simulink model "gm_HFMA_4B_1_5_9_13"  (R2026b)
settings: Solver=FixedStepDiscrete  StopTime=stopTime  FixedStep=1.953125e-06
PreLoadFcn:
  | load('a_luts.mat')
undefined symbols (not defined in the file or in its folder): Ts
libraries: simulink x202, simulink_need_slupdate x99, hdlsllib x91
(part 2 of 20)

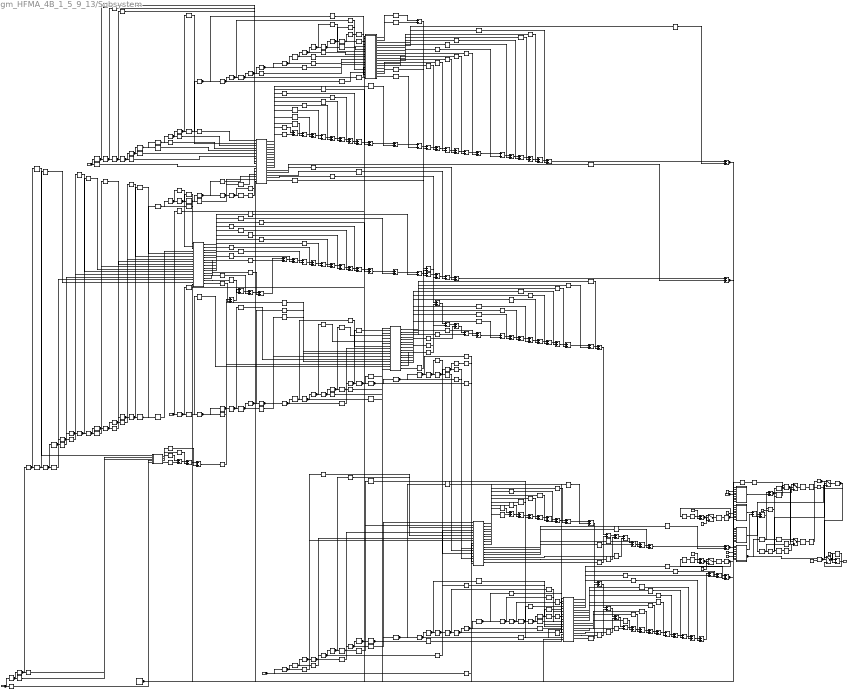
== system gm_HFMA_4B_1_5_9_13/Subsystem ==
  note: U(k)
  note: U(k)
  note: Latches the Output
  Mic1 : Inport  OutDataTypeStr=fixdt(1, 16, 15)  PortDimensions=1  SampleTime=0.000125
  Mic2 : Inport  Port=2  OutDataTypeStr=fixdt(1, 16, 15)  PortDimensions=1  SampleTime=0.000125
  Mic3 : Inport  Port=3  OutDataTypeStr=fixdt(1, 16, 15)  PortDimensions=1  SampleTime=0.000125
  Mic4 : Inport  Port=4  OutDataTypeStr=fixdt(1, 16, 15)  PortDimensions=1  SampleTime=0.000125
  RESET : Inport  Port=5  OutDataTypeStr=boolean  PortDimensions=1  SampleTime=0.000125
  Add{,25,27,29} (4 alike) : Sum  OutDataTypeStr=fixdt(1, 20, 17)  AccumDataTypeStr=fixdt(1, 22, 27)  SaturateOnIntegerOverflow=on  SampleTime=1.953125e-06
  Add{1,21,110,113,115,211..213} (8 alike) : Sum  OutDataTypeStr=fixdt(1, 20, 17)  AccumDataTypeStr=fixdt(1, 30, 26)  SaturateOnIntegerOverflow=on  SampleTime=1.953125e-06
  Add{7,10,12,15,71..73,101..103,121..123,151..153} (16 alike) : Sum  OutDataTypeStr=fixdt(1, 20, 17)  AccumDataTypeStr=fixdt(1, 24, 20)  SaturateOnIntegerOverflow=on  SampleTime=1.953125e-06
  Add{11,111..112,114} (4 alike) : Sum  OutDataTypeStr=fixdt(1, 20, 17)  AccumDataTypeStr=fixdt(1, 21, 17)  SaturateOnIntegerOverflow=on  SampleTime=1.953125e-06
  Add{9,13,91..93,131..133} (8 alike) : Sum  OutDataTypeStr=fixdt(1, 20, 17)  AccumDataTypeStr=fixdt(1, 23, 19)  SaturateOnIntegerOverflow=on  SampleTime=1.953125e-06
  Add{5,8,14,17,51..53,81..83,141..143,171..173} (16 alike) : Sum  OutDataTypeStr=fixdt(1, 20, 17)  AccumDataTypeStr=fixdt(1, 25, 21)  SaturateOnIntegerOverflow=on  SampleTime=1.953125e-06
  Add{2,6,16,20,24,26,28,61..63,161..163,201..203} (16 alike) : Sum  OutDataTypeStr=fixdt(1, 20, 17)  AccumDataTypeStr=fixdt(1, 27, 23)  SaturateOnIntegerOverflow=on  SampleTime=1.953125e-06
  Add{4,18,41..43,181..183} (8 alike) : Sum  OutDataTypeStr=fixdt(1, 20, 17)  AccumDataTypeStr=fixdt(1, 26, 22)  SaturateOnIntegerOverflow=on  SampleTime=1.953125e-06
  Add{3,19,22,31..33,191..193,221..223} (12 alike) : Sum  OutDataTypeStr=fixdt(1, 20, 17)  AccumDataTypeStr=fixdt(1, 28, 24)  SaturateOnIntegerOverflow=on  SampleTime=1.953125e-06
  Add{23,231..233} (4 alike) : Sum  OutDataTypeStr=fixdt(1, 20, 17)  AccumDataTypeStr=fixdt(1, 31, 27)  SaturateOnIntegerOverflow=on  SampleTime=1.953125e-06
  Add_stage2 : Sum  OutDataTypeStr=fixdt(0, 42, 34)  AccumDataTypeStr=fixdt(0, 42, 34)  SaturateOnIntegerOverflow=on  SampleTime=1.953125e-06
  Add_stage3 : Sum  OutDataTypeStr=fixdt(0, 42, 34)  AccumDataTypeStr=fixdt(0, 42, 34)  SaturateOnIntegerOverflow=on  SampleTime=1.953125e-06
  Add_stage4 : Sum  OutDataTypeStr=fixdt(0, 40, 34)  AccumDataTypeStr=fixdt(0, 42, 34)  SaturateOnIntegerOverflow=on  SampleTime=1.953125e-06
  Compare : RelationalOperator  Operator=<=  OutDataTypeStr=boolean  SampleTime=1.953125e-06
  Compare1 : RelationalOperator  Operator===  OutDataTypeStr=boolean  SampleTime=0.000125
  Constant : Constant  Value=0  OutDataTypeStr=uint8  SampleTime=1.953125e-06
  Constant1 : Constant  OutDataTypeStr=fixdt(0, 18, 0)  SampleTime=1.953125e-06
  Constant13 : Constant  Value=13  OutDataTypeStr=fixdt(0, 18, 0)  SampleTime=1.953125e-06
  Constant2 : Constant  Value=0  OutDataTypeStr=uint8  SampleTime=1.953125e-06
  Constant3 : Constant  Value=0  OutDataTypeStr=uint8  SampleTime=1.953125e-06
  Constant4 : Constant  Value=90  OutDataTypeStr=fixdt(0, 18, 11)  SampleTime=0.000125
  Constant5 : Constant  Value=5  OutDataTypeStr=fixdt(0, 18, 0)  SampleTime=1.953125e-06
  Constant6 : Constant  Value=180  OutDataTypeStr=uint8  SampleTime=0.000125
  Constant9 : Constant  Value=9  OutDataTypeStr=fixdt(0, 18, 0)  SampleTime=1.953125e-06
  Delay{,1..24,31..34,41..43,51..53,61..63,71..73,81..83,91..93,101..103,111..114,121..124,131..134,141..144,151..153,161..163,171..173,181..183,191..193,201..203,211..214,221..224,231..234} (96 alike) : Delay  DelayLength=1  InitialCondition=0  SampleTime=0.000125
  Delay110 : RateTransition  OutPortSampleTimeOpt=Multiple of input port sample time  OutPortSampleTimeMultiple=64
  Delay1_absorbed : Delay  DelayLength=0
  Delay25 : RateTransition  OutPortSampleTimeOpt=Multiple of input port sample time  OutPortSampleTimeMultiple=64
  Delay3_bypass : Delay  DelayLength=1  InitialCondition=0  SampleTime=0.000125
  Delay3_lowered : Delay  DelayLength=1  InitialCondition=0  SampleTime=0.000125
  Delay_Switch : Switch  Criteria=u2 ~= 0  OutDataTypeStr=uint8  SampleTime=0.000125  SaturateOnIntegerOverflow=off  InputSameDT=off
  Delay_absorbed : Delay  DelayLength=0
  FixPt Constant : Constant  OutDataTypeStr=uint8  SampleTime=1.953125e-06
  FixPt Constant1 : Constant  OutDataTypeStr=uint8  SampleTime=1.953125e-06
  FixPt Sum1 : Sum  OutDataTypeStr=uint8  AccumDataTypeStr=uint8  SampleTime=1.953125e-06
  FixPt Sum11 : Sum  OutDataTypeStr=uint8  AccumDataTypeStr=uint8  SampleTime=1.953125e-06
  FixPt Switch : Switch  Criteria=u2 > Threshold  Threshold="fi(0,0,8,0,\"hex\",\"27\")"  OutDataTypeStr=uint8  SampleTime=1.953125e-06  SaturateOnIntegerOverflow=off  InputSameDT=off
  FixPt Switch1 : Switch  Criteria=u2 > Threshold  Threshold="fi(0,0,8,0,\"hex\",\"b4\")"  OutDataTypeStr=uint8  SampleTime=1.953125e-06  SaturateOnIntegerOverflow=off  InputSameDT=off
  Force to be scalar : SignalSpecification  OutDataTypeStr=uint8  Dimensions=1
  Force to be scalar1 : SignalSpecification  OutDataTypeStr=uint8  Dimensions=1
  Gain10_out_dtc{,1..3} (4 alike) : DataTypeConversion  OutDataTypeStr=fixdt(1, 18, 19)  SampleTime=1.953125e-06  RndMeth=Floor
  Gain11_out_dtc{,1..3} (4 alike) : DataTypeConversion  OutDataTypeStr=fixdt(1, 18, 20)  SampleTime=1.953125e-06  RndMeth=Floor
  Gain12_out_dtc{,1..3} (4 alike) : DataTypeConversion  OutDataTypeStr=fixdt(1, 18, 17)  SampleTime=1.953125e-06  RndMeth=Floor
  Gain13_out_dtc{,1..3} (4 alike) : DataTypeConversion  OutDataTypeStr=fixdt(1, 18, 20)  SampleTime=1.953125e-06  RndMeth=Floor
  Gain14_out_dtc{,1..3} (4 alike) : DataTypeConversion  OutDataTypeStr=fixdt(1, 18, 19)  SampleTime=1.953125e-06  RndMeth=Floor
  Gain15_out_dtc{,1..3} (4 alike) : DataTypeConversion  OutDataTypeStr=fixdt(1, 18, 21)  SampleTime=1.953125e-06  RndMeth=Floor
  Gain16_out_dtc{,1..3} (4 alike) : DataTypeConversion  OutDataTypeStr=fixdt(1, 18, 20)  SampleTime=1.953125e-06  RndMeth=Floor
  Gain17_out_dtc{,1..3} (4 alike) : DataTypeConversion  OutDataTypeStr=fixdt(1, 18, 23)  SampleTime=1.953125e-06  RndMeth=Floor
  Gain18_out_dtc{,1..3} (4 alike) : DataTypeConversion  OutDataTypeStr=fixdt(1, 18, 21)  SampleTime=1.953125e-06  RndMeth=Floor
  Gain19_out_dtc{,1..3} (4 alike) : DataTypeConversion  OutDataTypeStr=fixdt(1, 18, 22)  SampleTime=1.953125e-06  RndMeth=Floor
  Gain1_out_dtc{,1..3} (4 alike) : DataTypeConversion  OutDataTypeStr=fixdt(1, 18, 24)  SampleTime=1.953125e-06  RndMeth=Floor
  Gain20_out_dtc{,1..3} (4 alike) : DataTypeConversion  OutDataTypeStr=fixdt(1, 18, 24)  SampleTime=1.953125e-06  RndMeth=Floor
  Gain21_out_dtc{,1..3} (4 alike) : DataTypeConversion  OutDataTypeStr=fixdt(1, 18, 23)  SampleTime=1.953125e-06  RndMeth=Floor
  Gain22_out_dtc{,1..3} (4 alike) : DataTypeConversion  OutDataTypeStr=fixdt(1, 18, 26)  SampleTime=1.953125e-06  RndMeth=Floor
  Gain23_out_dtc{,1..3} (4 alike) : DataTypeConversion  OutDataTypeStr=fixdt(1, 18, 24)  SampleTime=1.953125e-06  RndMeth=Floor
  Gain24_out_dtc{,1..3} (4 alike) : DataTypeConversion  OutDataTypeStr=fixdt(1, 18, 27)  SampleTime=1.953125e-06  RndMeth=Floor
  Gain2_out_dtc{,1..3} (4 alike) : DataTypeConversion  OutDataTypeStr=fixdt(1, 18, 26)  SampleTime=1.953125e-06  RndMeth=Floor
  Gain3_out_dtc{,1..3} (4 alike) : DataTypeConversion  OutDataTypeStr=fixdt(1, 18, 23)  SampleTime=1.953125e-06  RndMeth=Floor
  Gain4_out_dtc{,1..3} (4 alike) : DataTypeConversion  OutDataTypeStr=fixdt(1, 18, 24)  SampleTime=1.953125e-06  RndMeth=Floor
  Gain5_out_dtc{,1..3} (4 alike) : DataTypeConversion  OutDataTypeStr=fixdt(1, 18, 22)  SampleTime=1.953125e-06  RndMeth=Floor
  Gain6_out_dtc{,1..3} (4 alike) : DataTypeConversion  OutDataTypeStr=fixdt(1, 18, 21)  SampleTime=1.953125e-06  RndMeth=Floor
  Gain7_out_dtc{,1..3} (4 alike) : DataTypeConversion  OutDataTypeStr=fixdt(1, 18, 23)  SampleTime=1.953125e-06  RndMeth=Floor
  Gain8_out_dtc{,1..3} (4 alike) : DataTypeConversion  OutDataTypeStr=fixdt(1, 18, 20)  SampleTime=1.953125e-06  RndMeth=Floor
  Gain9_out_dtc{,1..3} (4 alike) : DataTypeConversion  OutDataTypeStr=fixdt(1, 18, 21)  SampleTime=1.953125e-06  RndMeth=Floor
  Gain_out_dtc{,1..3} (4 alike) : DataTypeConversion  OutDataTypeStr=fixdt(1, 18, 27)  SampleTime=1.953125e-06  RndMeth=Floor
  HFMA1 : Subsystem
  HFMA13 : Subsystem
  HFMA5 : Subsystem
  HFMA9 : Subsystem
  Logical Operator : Logic  Operator=OR  Inputs=3  AllPortsSameDT=off  OutDataTypeStr=boolean  SampleTime=1.953125e-06
  Output : Delay  DelayLength=1  InitialCondition=0  SampleTime=0.000125
  Output1 : Delay  DelayLength=1  InitialCondition=0  SampleTime=0.000125
  Output2 : RateTransition  OutPortSampleTimeOpt=Multiple of input port sample time  OutPortSampleTimeMultiple=64
  Output3 : RateTransition  OutPortSampleTimeOpt=Multiple of input port sample time  OutPortSampleTimeMultiple=64
  Relational Operator : RelationalOperator  Operator=>  OutDataTypeStr=boolean  SampleTime=1.953125e-06  InputSameDT=off
  Subtract : Sum  Inputs=+-  OutDataTypeStr=fixdt(1, 18, 10)  AccumDataTypeStr=fixdt(1, 20, 11)  SaturateOnIntegerOverflow=on  SampleTime=0.000125
  Switch : Switch  Criteria=u2 ~= 0  Threshold="fi(0,0,1,0,\"hex\",\"0\")"  OutDataTypeStr=fixdt(0, 40, 34)  SampleTime=1.953125e-06  SaturateOnIntegerOverflow=off  InputSameDT=off
  Switch1 : Switch  Criteria=u2 ~= 0  Threshold="fi(0,0,1,0,\"hex\",\"0\")"  OutDataTypeStr=uint8  SampleTime=1.953125e-06  SaturateOnIntegerOverflow=off  InputSameDT=off
  bypass_out : Switch  Criteria=u2 ~= 0  OutDataTypeStr=uint8  SampleTime=0.000125  SaturateOnIntegerOverflow=off  InputSameDT=off
  crp_out_delay : Delay  DelayLength=1  InitialCondition=0  SampleTime=1.953125e-06
  crp_out_delay1 : Delay  DelayLength=1  InitialCondition=0  SampleTime=1.953125e-06
  crp_temp_shared : Subsystem
  crp_temp_shared1 : Subsystem
  crp_temp_shared2 : Subsystem
  crp_temp_shared3 : Subsystem
  crp_temp_shared4 : Subsystem
  crp_temp_shared5 : Subsystem
  crp_temp_shared6 : Subsystem
  ctr_0_63 : hdlsllib/Sources/HDL Counter  CountType=Count limited  CountInit=0  CountStep=1  CountMax=63  CountFromType=Initial value  CountFrom=0  CountResetPort=off  CountLoadPort=off  CountEnbPort=off  CountDirPort=off  CountHitOutputPort=off  CountDataType=Unsigned  CountWordLen=6  CountFracLen=0  CountSampTime=1.953125e-06
  delayMatch : Delay  DelayLength=12  InitialCondition=0  SampleTime=1.953125e-06
  delayMatch{1..6} (6 alike) : Delay  DelayLength=1  InitialCondition=0  SampleTime=1.953125e-06
  in0_repeat : RateTransition  Integrity=off  Deterministic=off  OutPortSampleTimeOpt=Multiple of input port sample time  OutPortSampleTimeMultiple=1/64
  in0_repeat1 : RateTransition  Integrity=off  Deterministic=off  OutPortSampleTimeOpt=Multiple of input port sample time  OutPortSampleTimeMultiple=1/64
  in100_repeat : RateTransition  Integrity=off  Deterministic=off  OutPortSampleTimeOpt=Multiple of input port sample time  OutPortSampleTimeMultiple=1/64
  in101_repeat : RateTransition  Integrity=off  Deterministic=off  OutPortSampleTimeOpt=Multiple of input port sample time  OutPortSampleTimeMultiple=1/64
  in10_repeat : RateTransition  Integrity=off  Deterministic=off  OutPortSampleTimeOpt=Multiple of input port sample time  OutPortSampleTimeMultiple=1/64
  in11_repeat : RateTransition  Integrity=off  Deterministic=off  OutPortSampleTimeOpt=Multiple of input port sample time  OutPortSampleTimeMultiple=1/64
  in12_repeat : RateTransition  Integrity=off  Deterministic=off  OutPortSampleTimeOpt=Multiple of input port sample time  OutPortSampleTimeMultiple=1/64
  in13_repeat : RateTransition  Integrity=off  Deterministic=off  OutPortSampleTimeOpt=Multiple of input port sample time  OutPortSampleTimeMultiple=1/64
  in14_repeat : RateTransition  Integrity=off  Deterministic=off  OutPortSampleTimeOpt=Multiple of input port sample time  OutPortSampleTimeMultiple=1/64
  in15_repeat : RateTransition  Integrity=off  Deterministic=off  OutPortSampleTimeOpt=Multiple of input port sample time  OutPortSampleTimeMultiple=1/64
  in16_repeat : RateTransition  Integrity=off  Deterministic=off  OutPortSampleTimeOpt=Multiple of input port sample time  OutPortSampleTimeMultiple=1/64
  in17_repeat : RateTransition  Integrity=off  Deterministic=off  OutPortSampleTimeOpt=Multiple of input port sample time  OutPortSampleTimeMultiple=1/64
  in18_repeat : RateTransition  Integrity=off  Deterministic=off  OutPortSampleTimeOpt=Multiple of input port sample time  OutPortSampleTimeMultiple=1/64
  in19_repeat : RateTransition  Integrity=off  Deterministic=off  OutPortSampleTimeOpt=Multiple of input port sample time  OutPortSampleTimeMultiple=1/64
  in1_repeat : RateTransition  Integrity=off  Deterministic=off  OutPortSampleTimeOpt=Multiple of input port sample time  OutPortSampleTimeMultiple=1/64
  in1_repeat1 : RateTransition  Integrity=off  Deterministic=off  OutPortSampleTimeOpt=Multiple of input port sample time  OutPortSampleTimeMultiple=1/64
  in20_repeat : RateTransition  Integrity=off  Deterministic=off  OutPortSampleTimeOpt=Multiple of input port sample time  OutPortSampleTimeMultiple=1/64
  in21_repeat : RateTransition  Integrity=off  Deterministic=off  OutPortSampleTimeOpt=Multiple of input port sample time  OutPortSampleTimeMultiple=1/64
  in22_repeat : RateTransition  Integrity=off  Deterministic=off  OutPortSampleTimeOpt=Multiple of input port sample time  OutPortSampleTimeMultiple=1/64
  in23_repeat : RateTransition  Integrity=off  Deterministic=off  OutPortSampleTimeOpt=Multiple of input port sample time  OutPortSampleTimeMultiple=1/64
  in24_repeat : RateTransition  Integrity=off  Deterministic=off  OutPortSampleTimeOpt=Multiple of input port sample time  OutPortSampleTimeMultiple=1/64
  in25_repeat : RateTransition  Integrity=off  Deterministic=off  OutPortSampleTimeOpt=Multiple of input port sample time  OutPortSampleTimeMultiple=1/64
  in26_repeat : RateTransition  Integrity=off  Deterministic=off  OutPortSampleTimeOpt=Multiple of input port sample time  OutPortSampleTimeMultiple=1/64
  in27_repeat : RateTransition  Integrity=off  Deterministic=off  OutPortSampleTimeOpt=Multiple of input port sample time  OutPortSampleTimeMultiple=1/64
  in28_repeat : RateTransition  Integrity=off  Deterministic=off  OutPortSampleTimeOpt=Multiple of input port sample time  OutPortSampleTimeMultiple=1/64
  in29_repeat : RateTransition  Integrity=off  Deterministic=off  OutPortSampleTimeOpt=Multiple of input port sample time  OutPortSampleTimeMultiple=1/64
  in2_repeat : RateTransition  Integrity=off  Deterministic=off  OutPortSampleTimeOpt=Multiple of input port sample time  OutPortSampleTimeMultiple=1/64
  in2_repeat1 : RateTransition  Integrity=off  Deterministic=off  OutPortSampleTimeOpt=Multiple of input port sample time  OutPortSampleTimeMultiple=1/64
  in30_repeat : RateTransition  Integrity=off  Deterministic=off  OutPortSampleTimeOpt=Multiple of input port sample time  OutPortSampleTimeMultiple=1/64
  in31_repeat : RateTransition  Integrity=off  Deterministic=off  OutPortSampleTimeOpt=Multiple of input port sample time  OutPortSampleTimeMultiple=1/64
  in32_repeat : RateTransition  Integrity=off  Deterministic=off  OutPortSampleTimeOpt=Multiple of input port sample time  OutPortSampleTimeMultiple=1/64
  in33_repeat : RateTransition  Integrity=off  Deterministic=off  OutPortSampleTimeOpt=Multiple of input port sample time  OutPortSampleTimeMultiple=1/64
  in34_repeat : RateTransition  Integrity=off  Deterministic=off  OutPortSampleTimeOpt=Multiple of input port sample time  OutPortSampleTimeMultiple=1/64
  in35_repeat : RateTransition  Integrity=off  Deterministic=off  OutPortSampleTimeOpt=Multiple of input port sample time  OutPortSampleTimeMultiple=1/64
  in36_repeat : RateTransition  Integrity=off  Deterministic=off  OutPortSampleTimeOpt=Multiple of input port sample time  OutPortSampleTimeMultiple=1/64
  in37_repeat : RateTransition  Integrity=off  Deterministic=off  OutPortSampleTimeOpt=Multiple of input port sample time  OutPortSampleTimeMultiple=1/64
  in38_repeat : RateTransition  Integrity=off  Deterministic=off  OutPortSampleTimeOpt=Multiple of input port sample time  OutPortSampleTimeMultiple=1/64
  in39_repeat : RateTransition  Integrity=off  Deterministic=off  OutPortSampleTimeOpt=Multiple of input port sample time  OutPortSampleTimeMultiple=1/64
  in3_repeat : RateTransition  Integrity=off  Deterministic=off  OutPortSampleTimeOpt=Multiple of input port sample time  OutPortSampleTimeMultiple=1/64
  in3_repeat1 : RateTransition  Integrity=off  Deterministic=off  OutPortSampleTimeOpt=Multiple of input port sample time  OutPortSampleTimeMultiple=1/64
  in40_repeat : RateTransition  Integrity=off  Deterministic=off  OutPortSampleTimeOpt=Multiple of input port sample time  OutPortSampleTimeMultiple=1/64
  in41_repeat : RateTransition  Integrity=off  Deterministic=off  OutPortSampleTimeOpt=Multiple of input port sample time  OutPortSampleTimeMultiple=1/64
  in42_repeat : RateTransition  Integrity=off  Deterministic=off  OutPortSampleTimeOpt=Multiple of input port sample time  OutPortSampleTimeMultiple=1/64
  in43_repeat : RateTransition  Integrity=off  Deterministic=off  OutPortSampleTimeOpt=Multiple of input port sample time  OutPortSampleTimeMultiple=1/64
  in44_repeat : RateTransition  Integrity=off  Deterministic=off  OutPortSampleTimeOpt=Multiple of input port sample time  OutPortSampleTimeMultiple=1/64
  in45_repeat : RateTransition  Integrity=off  Deterministic=off  OutPortSampleTimeOpt=Multiple of input port sample time  OutPortSampleTimeMultiple=1/64
  in46_repeat : RateTransition  Integrity=off  Deterministic=off  OutPortSampleTimeOpt=Multiple of input port sample time  OutPortSampleTimeMultiple=1/64
  in47_repeat : RateTransition  Integrity=off  Deterministic=off  OutPortSampleTimeOpt=Multiple of input port sample time  OutPortSampleTimeMultiple=1/64
  in48_repeat : RateTransition  Integrity=off  Deterministic=off  OutPortSampleTimeOpt=Multiple of input port sample time  OutPortSampleTimeMultiple=1/64
  in49_repeat : RateTransition  Integrity=off  Deterministic=off  OutPortSampleTimeOpt=Multiple of input port sample time  OutPortSampleTimeMultiple=1/64
  in4_repeat : RateTransition  Integrity=off  Deterministic=off  OutPortSampleTimeOpt=Multiple of input port sample time  OutPortSampleTimeMultiple=1/64
  in50_repeat : RateTransition  Integrity=off  Deterministic=off  OutPortSampleTimeOpt=Multiple of input port sample time  OutPortSampleTimeMultiple=1/64
  in51_repeat : RateTransition  Integrity=off  Deterministic=off  OutPortSampleTimeOpt=Multiple of input port sample time  OutPortSampleTimeMultiple=1/64
  in52_repeat : RateTransition  Integrity=off  Deterministic=off  OutPortSampleTimeOpt=Multiple of input port sample time  OutPortSampleTimeMultiple=1/64
  in53_repeat : RateTransition  Integrity=off  Deterministic=off  OutPortSampleTimeOpt=Multiple of input port sample time  OutPortSampleTimeMultiple=1/64
  in54_repeat : RateTransition  Integrity=off  Deterministic=off  OutPortSampleTimeOpt=Multiple of input port sample time  OutPortSampleTimeMultiple=1/64
  in55_repeat : RateTransition  Integrity=off  Deterministic=off  OutPortSampleTimeOpt=Multiple of input port sample time  OutPortSampleTimeMultiple=1/64
  in56_repeat : RateTransition  Integrity=off  Deterministic=off  OutPortSampleTimeOpt=Multiple of input port sample time  OutPortSampleTimeMultiple=1/64
  in57_repeat : RateTransition  Integrity=off  Deterministic=off  OutPortSampleTimeOpt=Multiple of input port sample time  OutPortSampleTimeMultiple=1/64
  in58_repeat : RateTransition  Integrity=off  Deterministic=off  OutPortSampleTimeOpt=Multiple of input port sample time  OutPortSampleTimeMultiple=1/64
  in59_repeat : RateTransition  Integrity=off  Deterministic=off  OutPortSampleTimeOpt=Multiple of input port sample time  OutPortSampleTimeMultiple=1/64
  in5_repeat : RateTransition  Integrity=off  Deterministic=off  OutPortSampleTimeOpt=Multiple of input port sample time  OutPortSampleTimeMultiple=1/64
  in60_repeat : RateTransition  Integrity=off  Deterministic=off  OutPortSampleTimeOpt=Multiple of input port sample time  OutPortSampleTimeMultiple=1/64
  in61_repeat : RateTransition  Integrity=off  Deterministic=off  OutPortSampleTimeOpt=Multiple of input port sample time  OutPortSampleTimeMultiple=1/64
  in62_repeat : RateTransition  Integrity=off  Deterministic=off  OutPortSampleTimeOpt=Multiple of input port sample time  OutPortSampleTimeMultiple=1/64
  in63_repeat : RateTransition  Integrity=off  Deterministic=off  OutPortSampleTimeOpt=Multiple of input port sample time  OutPortSampleTimeMultiple=1/64
  in64_repeat : RateTransition  Integrity=off  Deterministic=off  OutPortSampleTimeOpt=Multiple of input port sample time  OutPortSampleTimeMultiple=1/64
  in65_repeat : RateTransition  Integrity=off  Deterministic=off  OutPortSampleTimeOpt=Multiple of input port sample time  OutPortSampleTimeMultiple=1/64
  in66_repeat : RateTransition  Integrity=off  Deterministic=off  OutPortSampleTimeOpt=Multiple of input port sample time  OutPortSampleTimeMultiple=1/64
  in67_repeat : RateTransition  Integrity=off  Deterministic=off  OutPortSampleTimeOpt=Multiple of input port sample time  OutPortSampleTimeMultiple=1/64
  in68_repeat : RateTransition  Integrity=off  Deterministic=off  OutPortSampleTimeOpt=Multiple of input port sample time  OutPortSampleTimeMultiple=1/64
  in69_repeat : RateTransition  Integrity=off  Deterministic=off  OutPortSampleTimeOpt=Multiple of input port sample time  OutPortSampleTimeMultiple=1/64
  in6_repeat : RateTransition  Integrity=off  Deterministic=off  OutPortSampleTimeOpt=Multiple of input port sample time  OutPortSampleTimeMultiple=1/64
  in70_repeat : RateTransition  Integrity=off  Deterministic=off  OutPortSampleTimeOpt=Multiple of input port sample time  OutPortSampleTimeMultiple=1/64
  in71_repeat : RateTransition  Integrity=off  Deterministic=off  OutPortSampleTimeOpt=Multiple of input port sample time  OutPortSampleTimeMultiple=1/64
  in72_repeat : RateTransition  Integrity=off  Deterministic=off  OutPortSampleTimeOpt=Multiple of input port sample time  OutPortSampleTimeMultiple=1/64
  in73_repeat : RateTransition  Integrity=off  Deterministic=off  OutPortSampleTimeOpt=Multiple of input port sample time  OutPortSampleTimeMultiple=1/64
  in74_repeat : RateTransition  Integrity=off  Deterministic=off  OutPortSampleTimeOpt=Multiple of input port sample time  OutPortSampleTimeMultiple=1/64
  in75_repeat : RateTransition  Integrity=off  Deterministic=off  OutPortSampleTimeOpt=Multiple of input port sample time  OutPortSampleTimeMultiple=1/64
  in76_repeat : RateTransition  Integrity=off  Deterministic=off  OutPortSampleTimeOpt=Multiple of input port sample time  OutPortSampleTimeMultiple=1/64
  in77_repeat : RateTransition  Integrity=off  Deterministic=off  OutPortSampleTimeOpt=Multiple of input port sample time  OutPortSampleTimeMultiple=1/64
  in78_repeat : RateTransition  Integrity=off  Deterministic=off  OutPortSampleTimeOpt=Multiple of input port sample time  OutPortSampleTimeMultiple=1/64
  in79_repeat : RateTransition  Integrity=off  Deterministic=off  OutPortSampleTimeOpt=Multiple of input port sample time  OutPortSampleTimeMultiple=1/64
  in7_repeat : RateTransition  Integrity=off  Deterministic=off  OutPortSampleTimeOpt=Multiple of input port sample time  OutPortSampleTimeMultiple=1/64
  in80_repeat : RateTransition  Integrity=off  Deterministic=off  OutPortSampleTimeOpt=Multiple of input port sample time  OutPortSampleTimeMultiple=1/64
  in81_repeat : RateTransition  Integrity=off  Deterministic=off  OutPortSampleTimeOpt=Multiple of input port sample time  OutPortSampleTimeMultiple=1/64
  in82_repeat : RateTransition  Integrity=off  Deterministic=off  OutPortSampleTimeOpt=Multiple of input port sample time  OutPortSampleTimeMultiple=1/64
  in83_repeat : RateTransition  Integrity=off  Deterministic=off  OutPortSampleTimeOpt=Multiple of input port sample time  OutPortSampleTimeMultiple=1/64
  in84_repeat : RateTransition  Integrity=off  Deterministic=off  OutPortSampleTimeOpt=Multiple of input port sample time  OutPortSampleTimeMultiple=1/64
  in85_repeat : RateTransition  Integrity=off  Deterministic=off  OutPortSampleTimeOpt=Multiple of input port sample time  OutPortSampleTimeMultiple=1/64
  in86_repeat : RateTransition  Integrity=off  Deterministic=off  OutPortSampleTimeOpt=Multiple of input port sample time  OutPortSampleTimeMultiple=1/64
  in87_repeat : RateTransition  Integrity=off  Deterministic=off  OutPortSampleTimeOpt=Multiple of input port sample time  OutPortSampleTimeMultiple=1/64
  in88_repeat : RateTransition  Integrity=off  Deterministic=off  OutPortSampleTimeOpt=Multiple of input port sample time  OutPortSampleTimeMultiple=1/64
  in89_repeat : RateTransition  Integrity=off  Deterministic=off  OutPortSampleTimeOpt=Multiple of input port sample time  OutPortSampleTimeMultiple=1/64
  in8_repeat : RateTransition  Integrity=off  Deterministic=off  OutPortSampleTimeOpt=Multiple of input port sample time  OutPortSampleTimeMultiple=1/64
  in90_repeat : RateTransition  Integrity=off  Deterministic=off  OutPortSampleTimeOpt=Multiple of input port sample time  OutPortSampleTimeMultiple=1/64
  in91_repeat : RateTransition  Integrity=off  Deterministic=off  OutPortSampleTimeOpt=Multiple of input port sample time  OutPortSampleTimeMultiple=1/64
  in92_repeat : RateTransition  Integrity=off  Deterministic=off  OutPortSampleTimeOpt=Multiple of input port sample time  OutPortSampleTimeMultiple=1/64
  in93_repeat : RateTransition  Integrity=off  Deterministic=off  OutPortSampleTimeOpt=Multiple of input port sample time  OutPortSampleTimeMultiple=1/64
  in94_repeat : RateTransition  Integrity=off  Deterministic=off  OutPortSampleTimeOpt=Multiple of input port sample time  OutPortSampleTimeMultiple=1/64
  in95_repeat : RateTransition  Integrity=off  Deterministic=off  OutPortSampleTimeOpt=Multiple of input port sample time  OutPortSampleTimeMultiple=1/64
  in96_repeat : RateTransition  Integrity=off  Deterministic=off  OutPortSampleTimeOpt=Multiple of input port sample time  OutPortSampleTimeMultiple=1/64
  in97_repeat : RateTransition  Integrity=off  Deterministic=off  OutPortSampleTimeOpt=Multiple of input port sample time  OutPortSampleTimeMultiple=1/64
  in98_repeat : RateTransition  Integrity=off  Deterministic=off  OutPortSampleTimeOpt=Multiple of input port sample time  OutPortSampleTimeMultiple=1/64
  in99_repeat : RateTransition  Integrity=off  Deterministic=off  OutPortSampleTimeOpt=Multiple of input port sample time  OutPortSampleTimeMultiple=1/64
  in9_repeat : RateTransition  Integrity=off  Deterministic=off  OutPortSampleTimeOpt=Multiple of input port sample time  OutPortSampleTimeMultiple=1/64
  DOA : Outport  OutDataTypeStr=fixdt(1, 18, 10)  PortDimensions=1  SampleTime=0.000125
  wires:
  crp_temp_shared6/4(out3) -> Gain_out_dtc3/1
  Add22/1 -> Add23/1
  delayMatch1/1 -> Relational Operator/2
  in32_repeat/1 -> crp_temp_shared2/1(in0)
  crp_temp_shared3/1(out0) -> Gain1_out_dtc1/1
  Add115/1 -> Add28/1
  Add21/1 -> Add22/1
  Add28/1 -> delayMatch/1
  Relational Operator/1 -> Logical Operator/1
  Add93/1 -> Add103/1
  Switch1/1 -> crp_out_delay1/1
  Add83/1 -> Add93/1
  Delay10/1 -> in38_repeat/1, Delay111/1
  in19_repeat/1 -> crp_temp_shared1/4(in3)
  Compare/1 -> delayMatch3/1
  Add103/1 -> Add114/1
  Delay93/1 -> in14_repeat/1, Delay103/1
  Delay92/1 -> in89_repeat/1, Delay102/1
  Gain9_out_dtc2/1 -> Add82/2
  Add14/1 -> Add15/1
  crp_temp_shared1/7(out6) -> Gain2_out_dtc/1
  crp_temp_shared1/9(out8) -> Gain_out_dtc/1
  crp_temp_shared6/1(out0) -> Gain3_out_dtc3/1
  Gain14_out_dtc3/1 -> Add133/2
  Add2/1 -> Add3/1
  crp_temp_shared2/12(out11) -> Gain6_out_dtc1/1
  Switch/1 -> crp_out_delay/1
  Gain13_out_dtc2/1 -> Add122/2
  Add_stage3/1 -> Add_stage4/1
  in25_repeat/1 -> crp_temp_shared1/10(in9)
  Add4/1 -> Add5/1
  Add_stage2/1 -> Add_stage3/1
  delayMatch6/1 -> Switch1/3
  in35_repeat/1 -> crp_temp_shared2/4(in3)
  Delay142/1 -> in59_repeat/1, Delay151/1
  in8_repeat/1 -> crp_temp_shared/9(in8)
  Add72/1 -> Add82/1
  delayMatch4/1 -> Switch/3
  Delay191/1 -> in54_repeat/1, Delay201/1
  Delay34/1 -> in20_repeat/1, Delay43/1
  Add26/1 -> Add32/1
  crp_temp_shared4/3(out2) -> Gain8_out_dtc2/1
  Add27/1 -> Add113/1
  in84_repeat/1 -> crp_temp_shared5/5(in4)
  Delay43/1 -> in19_repeat/1, Delay53/1
  Add113/1 -> Add26/1
  Delay224/1 -> Delay234/1, in1_repeat/1
  in72_repeat/1 -> crp_temp_shared4/9(in8)
  in24_repeat/1 -> crp_temp_shared1/9(in8)
  HFMA5/1(P_theta) -> Add_stage2/2
  Add153/1 -> Add163/1
  Gain12_out_dtc2/1 -> Add112/2
  Add212/1 -> Add222/1
  Gain9_out_dtc3/1 -> Add83/2
  Add133/1 -> Add143/1
  delayMatch3/1 -> Logical Operator/3
  Delay144/1 -> in9_repeat/1, Delay153/1
  Constant3/1 -> Compare/2
  in22_repeat/1 -> crp_temp_shared1/7(in6)
  Delay103/1 -> in13_repeat/1, Delay114/1
  Delay52/1 -> in93_repeat/1, Delay62/1
  crp_temp_shared/3(out2) -> Gain22_out_dtc/1
  Add31/1 -> Add41/1
  crp_temp_shared3/7(out6) -> Gain20_out_dtc2/1
  in61_repeat/1 -> crp_temp_shared3/14(in13)
  crp_temp_shared3/11(out10) -> Gain16_out_dtc2/1
  in4_repeat/1 -> crp_temp_shared/5(in4)
  Gain1_out_dtc/1 -> Add/1
  Add111/1 -> Add121/1
  bypass_out/1 -> Subtract/1, Delay3_bypass/1
  Add91/1 -> Add101/1
  Mic3/1 -> in74_repeat/1, Delay1/1
  crp_temp_shared3/16(out15) -> Gain11_out_dtc2/1
  crp_temp_shared/16(out15) -> Gain9_out_dtc/1
  in101_repeat/1 -> Force to be scalar1/1
  in31_repeat/1 -> crp_temp_shared1/16(in15)
  delayMatch2/1 -> Logical Operator/2
  crp_temp_shared4/15(out14) -> Gain21_out_dtc3/1
  crp_temp_shared6/3(out2) -> Gain1_out_dtc3/1
  crp_temp_shared4/11(out10) -> Gain_out_dtc2/1
  crp_temp_shared5/14(out13) -> Gain6_out_dtc3/1
  crp_temp_shared4/5(out4) -> Gain6_out_dtc2/1
  in78_repeat/1 -> crp_temp_shared4/15(in14)
  Gain22_out_dtc3/1 -> Add213/2
  Output/1 -> in100_repeat/1, HFMA13/7(IQ Counter), HFMA5/7(IQ Counter), HFMA9/7(IQ Counter), HFMA1/7(IQ Counter)
  Gain2_out_dtc3/1 -> Add115/2
  crp_temp_shared5/16(out15) -> Gain4_out_dtc3/1
  Delay4/1 -> in44_repeat/1, Delay5/1
  Gain2_out_dtc1/1 -> Add110/2
  crp_temp_shared5/9(out8) -> Gain11_out_dtc3/1
  crp_temp_shared/9(out8) -> Gain16_out_dtc/1
  crp_temp_shared4/4(out3) -> Gain7_out_dtc2/1
  in88_repeat/1 -> crp_temp_shared5/9(in8)
  Gain10_out_dtc1/1 -> Add91/2
  crp_temp_shared5/4(out3) -> Gain16_out_dtc3/1
  Delay141/1 -> in34_repeat/1, Delay15/1
  Delay183/1 -> in5_repeat/1, Delay193/1
  Delay32/1 -> in70_repeat/1, Delay41/1
  Add162/1 -> Add172/1
  Gain22_out_dtc1/1 -> Add211/2
  Delay181/1 -> in55_repeat/1, Delay191/1
  crp_temp_shared3/15(out14) -> Gain12_out_dtc2/1
  Delay3/1 -> in23_repeat/1, Delay14/1
  crp_temp_shared4/10(out9) -> Gain1_out_dtc2/1
  Gain17_out_dtc2/1 -> Add162/2
  crp_temp_shared2/8(out7) -> Gain10_out_dtc1/1
  in90_repeat/1 -> crp_temp_shared5/11(in10)
  Add18/1 -> Add19/1
  Delay143/1 -> Delay152/1, in84_repeat/1
  Constant2/1 -> FixPt Switch1/1
  crp_out_delay/1 -> Delay25/1
  crp_temp_shared3/8(out7) -> Gain19_out_dtc2/1
  Add231/1 -> HFMA1/2(Mic2), HFMA9/2(Mic2), HFMA5/2(Mic2), HFMA13/2(Mic2)
  Delay111/1 -> in37_repeat/1, Delay121/1
  Force to be scalar1/1 -> FixPt Sum11/1
  Gain2_out_dtc2/1 -> Add113/2
  crp_temp_shared3/5(out4) -> Gain22_out_dtc2/1
  Add102/1 -> Add112/1
  Add151/1 -> Add161/1
  in75_repeat/1 -> crp_temp_shared4/12(in11)
  crp_temp_shared4/7(out6) -> Gain4_out_dtc2/1
  crp_temp_shared3/2(out1) -> Gain_out_dtc1/1
  Delay122/1 -> Delay132/1, in61_repeat/1
  Gain18_out_dtc3/1 -> Add173/2
  crp_temp_shared2/16(out15) -> Gain2_out_dtc1/1
  Delay172/1 -> Delay182/1, in81_repeat/1
  Add5/1 -> Add6/1
  Add/1 -> Add1/1
  Gain1_out_dtc2/1 -> Add27/1
  Add132/1 -> Add142/1
  Add152/1 -> Add162/1
  Gain18_out_dtc1/1 -> Add171/2
  Add23/1 -> HFMA13/1(Mic1), HFMA5/1(Mic1), HFMA1/1(Mic1), HFMA9/1(Mic1)
  Add9/1 -> Add10/1
  in59_repeat/1 -> crp_temp_shared3/12(in11)
  in80_repeat/1 -> crp_temp_shared5/1(in0)
  in11_repeat/1 -> crp_temp_shared/12(in11)
  Gain16_out_dtc2/1 -> Add152/2
  Add183/1 -> Add193/1
  Add172/1 -> Add182/1
  Delay214/1 -> Delay224/1, in2_repeat/1
  Gain15_out_dtc/1 -> Add14/2
  Output1/1 -> in101_repeat/1, HFMA13/8(A Counter), HFMA9/8(A Counter), HFMA5/8(A Counter), HFMA1/8(A Counter)
  Gain8_out_dtc/1 -> Add7/2
  Add8/1 -> Add9/1
  Constant6/1 -> Compare1/2
  Add101/1 -> Add111/1
  crp_temp_shared1/8(out7) -> Gain1_out_dtc/1
  Delay71/1 -> in66_repeat/1, Delay81/1
  crp_out_delay1/1 -> Delay110/1
  Add82/1 -> Add92/1
  in3_repeat1/1 -> delayMatch2/1
  Add110/1 -> Add24/1
  Mic4/1 -> in99_repeat/1, Delay2/1
  Add192/1 -> Add202/1
  Gain10_out_dtc/1 -> Add9/2
  Add81/1 -> Add91/1
  crp_temp_shared4/2(out1) -> Gain9_out_dtc2/1
  Delay33/1 -> Delay42/1, in95_repeat/1
  Gain17_out_dtc/1 -> Add16/2
  Delay161/1 -> in57_repeat/1, Delay171/1
  delayMatch/1 -> Add33/1
  FixPt Constant1/1 -> FixPt Sum11/2
  crp_temp_shared4/14(out13) -> Gain22_out_dtc3/1
  Gain13_out_dtc1/1 -> Add121/2
  FixPt Constant/1 -> FixPt Sum1/2
  Delay231/1 -> in25_repeat/1
  in73_repeat/1 -> crp_temp_shared4/10(in9)
  Force to be scalar/1 -> FixPt Sum1/1
  Constant/1 -> FixPt Switch/1
  Delay13/1 -> Delay23/1, in97_repeat/1
  Gain10_out_dtc2/1 -> Add92/2
  Delay162/1 -> in82_repeat/1, Delay172/1
  crp_temp_shared2/3(out2) -> Gain15_out_dtc1/1
  ctr_0_63/1 -> HFMA13/9(sch_ctr_63), crp_temp_shared4/17(enb_counter), HFMA9/9(sch_ctr_63), crp_temp_shared2/17(enb_counter), crp_temp_shared3/17(enb_counter), crp_temp_shared/17(enb_counter), HFMA5/9(sch_ctr_63), HFMA1/9(sch_ctr_63), crp_temp_shared5/17(enb_counter), crp_temp_shared6/5(enb_counter), crp_temp_shared1/17(enb_counter)
  crp_temp_shared1/16(out15) -> Gain18_out_dtc1/1
  Add29/1 -> Add115/1
  Delay22/1 -> Delay32/1, in71_repeat/1
  Gain5_out_dtc/1 -> Add4/2
  Gain_out_dtc3/1 -> Add29/2
  HFMA9/1(P_theta) -> Add_stage3/2
  Gain1_out_dtc3/1 -> Add29/1
  Add33/1 -> Add43/1
  Delay123/1 -> Delay133/1, in86_repeat/1
  Add61/1 -> Add71/1
  Gain21_out_dtc3/1 -> Add203/2
  Delay171/1 -> in56_repeat/1, Delay181/1
  Gain4_out_dtc3/1 -> Add33/2
  Gain13_out_dtc/1 -> Add12/2
  Add43/1 -> Add53/1
  Delay113/1 -> Delay123/1, in87_repeat/1
  Delay3_bypass/1 -> bypass_out/3
  Gain5_out_dtc3/1 -> Add43/2
  Add182/1 -> Add192/1
  Add53/1 -> Add63/1
  Gain21_out_dtc2/1 -> Add202/2
  Add63/1 -> Add73/1
  Gain_out_dtc2/1 -> Add27/2
  Gain7_out_dtc3/1 -> Add63/2
  in10_repeat/1 -> crp_temp_shared/11(in10)
  Add73/1 -> Add83/1
  Gain8_out_dtc3/1 -> Add73/2
  Add15/1 -> Add16/1
  in23_repeat/1 -> crp_temp_shared1/8(in7)
  Add114/1 -> Add123/1
  Delay163/1 -> in7_repeat/1, Delay173/1
  Add123/1 -> Add133/1
  Add25/1 -> Add110/1
  Add222/1 -> Add232/1
  Add232/1 -> HFMA1/3(Mic3), HFMA13/3(Mic3), HFMA5/3(Mic3), HFMA9/3(Mic3)
  Delay131/1 -> Delay141/1, in35_repeat/1
  Delay124/1 -> in11_repeat/1, Delay134/1
  Mic2/1 -> Delay/1, in49_repeat/1
  Add_stage4/1 -> Switch/1, Relational Operator/1
  Add143/1 -> Add153/1
  Gain13_out_dtc3/1 -> Add123/2
  Gain24_out_dtc/1 -> Add23/2
  Delay110/1 -> Delay1_absorbed/1
  in44_repeat/1 -> crp_temp_shared2/13(in12)
  Add13/1 -> Add14/1
  Delay21/1 -> in46_repeat/1, Delay31/1
  in27_repeat/1 -> crp_temp_shared1/12(in11)
  Add163/1 -> Add173/1
  in96_repeat/1 -> crp_temp_shared6/1(in0)
  crp_temp_shared2/7(out6) -> Gain11_out_dtc1/1
  Add173/1 -> Add183/1
  in45_repeat/1 -> crp_temp_shared2/14(in13)
  FixPt Switch/1 -> Output2/1
  crp_temp_shared1/6(out5) -> Gain3_out_dtc/1
  Gain19_out_dtc3/1 -> Add183/2
  Delay153/1 -> in8_repeat/1, Delay163/1
  crp_temp_shared2/15(out14) -> Gain3_out_dtc1/1
  Gain21_out_dtc/1 -> Add20/2
  in41_repeat/1 -> crp_temp_shared2/10(in9)
  Add193/1 -> Add203/1
  Delay62/1 -> Delay72/1, in92_repeat/1
  Delay221/1 -> in26_repeat/1, Delay231/1
  Delay114/1 -> in12_repeat/1, Delay124/1
  Add203/1 -> Add213/1
  Add20/1 -> Add21/1
  crp_temp_shared5/6(out5) -> Gain14_out_dtc3/1
  Gain12_out_dtc1/1 -> Add111/2
  in7_repeat/1 -> crp_temp_shared/8(in7)
  Add213/1 -> Add223/1
  Gain7_out_dtc1/1 -> Add61/2
  Add62/1 -> Add72/1
  Constant9/1 -> HFMA9/6(F0 Index)
  in97_repeat/1 -> crp_temp_shared6/2(in1)
  Gain3_out_dtc2/1 -> Add26/2
  Add233/1 -> HFMA13/4(Mic4), HFMA9/4(Mic4), HFMA1/4(Mic4), HFMA5/4(Mic4)
  Add161/1 -> Add171/1
  Add32/1 -> Add42/1
  Gain3_out_dtc1/1 -> Add24/2
  Constant13/1 -> HFMA13/6(F0 Index)
  Delay11/1 -> in47_repeat/1, Delay21/1
  in9_repeat/1 -> crp_temp_shared/10(in9)
  Subtract/1 -> DOA/1
  in51_repeat/1 -> crp_temp_shared3/4(in3)
  Add42/1 -> Add52/1
  Add52/1 -> Add62/1
  Delay83/1 -> Delay93/1, in15_repeat/1
  Add92/1 -> Add102/1
  Add10/1 -> Add11/1
  Delay23/1 -> in96_repeat/1, Delay33/1
  in38_repeat/1 -> crp_temp_shared2/7(in6)
  Delay223/1 -> in76_repeat/1, Delay233/1
  Gain11_out_dtc2/1 -> Add102/2
  Add112/1 -> Add122/1
  Add122/1 -> Add132/1
  Gain14_out_dtc2/1 -> Add132/2
  HFMA5/2(Theta) -> Compare1/1, in0_repeat1/1
  in26_repeat/1 -> crp_temp_shared1/11(in10)
  crp_temp_shared4/8(out7) -> Gain3_out_dtc2/1
  crp_temp_shared3/3(out2) -> Gain24_out_dtc2/1
  Add142/1 -> Add152/1
  in81_repeat/1 -> crp_temp_shared5/2(in1)
  Gain15_out_dtc2/1 -> Add142/2
  Delay42/1 -> in94_repeat/1, Delay52/1
  crp_temp_shared/11(out10) -> Gain14_out_dtc/1
  Delay1/1 -> Delay12/1, in73_repeat/1
  Gain10_out_dtc3/1 -> Add93/2
  Add3/1 -> Add4/1
  Add202/1 -> Add212/1
  Output2/1 -> Output/1
  in13_repeat/1 -> crp_temp_shared/14(in13)
  Gain_out_dtc1/1 -> Add25/2
  Gain22_out_dtc2/1 -> Add212/2
  Compare1/1 -> Delay_Switch/2, bypass_out/2
  Gain11_out_dtc/1 -> Add10/2
  Gain1_out_dtc1/1 -> Add25/1
  Delay151/1 -> in58_repeat/1, Delay161/1
  Add24/1 -> Add31/1
  Gain23_out_dtc/1 -> Add22/2
  Add41/1 -> Add51/1
  in0_repeat1/1 -> delayMatch5/1, Compare/1
  in43_repeat/1 -> crp_temp_shared2/12(in11)
  Add121/1 -> Add131/1
  Delay202/1 -> Delay213/1, in78_repeat/1
  Add51/1 -> Add61/1
  Add71/1 -> Add81/1
  Add19/1 -> Add20/1
  Gain8_out_dtc1/1 -> Add71/2
  in60_repeat/1 -> crp_temp_shared3/13(in12)
  crp_temp_shared1/3(out2) -> Gain6_out_dtc/1
  Add7/1 -> Add8/1
  Gain15_out_dtc1/1 -> Add141/2
  Add131/1 -> Add141/1
  Delay232/1 -> in50_repeat/1
  crp_temp_shared/1(out0) -> Gain24_out_dtc/1
  Delay5/1 -> in43_repeat/1, Delay6/1
  Add141/1 -> Add151/1
  Gain16_out_dtc1/1 -> Add151/2
  in76_repeat/1 -> crp_temp_shared4/13(in12)
  Gain17_out_dtc1/1 -> Add161/2
  crp_temp_shared3/6(out5) -> Gain21_out_dtc2/1
  Add171/1 -> Add181/1
  Add191/1 -> Add201/1
  Add181/1 -> Add191/1
  Gain19_out_dtc1/1 -> Add181/2
  Add201/1 -> Add211/1
  Gain20_out_dtc1/1 -> Add191/2
  Constant4/1 -> Subtract/2
  Add211/1 -> Add221/1
  Delay112/1 -> in62_repeat/1, Delay122/1
  Constant5/1 -> HFMA5/6(F0 Index)
  Delay193/1 -> in4_repeat/1, Delay203/1
  Delay12/1 -> in72_repeat/1, Delay22/1
  crp_temp_shared3/13(out12) -> Gain14_out_dtc2/1
  Delay121/1 -> Delay131/1, in36_repeat/1
  Gain_out_dtc/1 -> Add/2
  Add1/1 -> Add2/1
  Delay192/1 -> Delay202/1, in79_repeat/1
  FixPt Sum1/1 -> FixPt Switch/2, FixPt Switch/3
  Gain2_out_dtc/1 -> Add1/2
  Gain3_out_dtc/1 -> Add2/2
  crp_temp_shared/14(out13) -> Gain11_out_dtc/1
  Gain4_out_dtc/1 -> Add3/2
  Delay2/1 -> Delay13/1, in98_repeat/1
  HFMA13/1(P_theta) -> Add_stage4/2
  Add6/1 -> Add7/1
  Gain7_out_dtc/1 -> Add6/2
  Gain9_out_dtc/1 -> Add8/2
  Add11/1 -> Add12/1
  Gain12_out_dtc/1 -> Add11/2
  Add12/1 -> Add13/1
  in89_repeat/1 -> crp_temp_shared5/10(in9)
  Delay134/1 -> in10_repeat/1, Delay144/1
  Gain14_out_dtc/1 -> Add13/2
  Delay201/1 -> in53_repeat/1, Delay212/1
  Gain16_out_dtc/1 -> Add15/2
  Delay17/1 -> in31_repeat/1, Delay18/1
  Gain20_out_dtc/1 -> Add19/2
  in40_repeat/1 -> crp_temp_shared2/9(in8)
  Add16/1 -> Add17/1
  Delay6/1 -> in42_repeat/1, Delay7/1
  Add17/1 -> Add18/1
  Delay133/1 -> in85_repeat/1, Delay143/1
  Delay25/1 -> Delay_absorbed/1
  in1_repeat1/1 -> delayMatch6/1
  Output3/1 -> Output1/1
  Mic1/1 -> in24_repeat/1, Delay3/1
  Gain6_out_dtc2/1 -> Add52/2
  FixPt Switch1/1 -> Output3/1
  RESET/1 -> HFMA5/5(RESET), HFMA13/5(RESET), in3_repeat1/1, HFMA9/5(RESET), HFMA1/5(RESET)
  in100_repeat/1 -> Force to be scalar/1
  in49_repeat/1 -> crp_temp_shared3/2(in1)
  Delay234/1 -> in0_repeat/1
  Delay1_absorbed/1 -> in1_repeat1/1, Delay_Switch/1
  Delay53/1 -> in18_repeat/1, Delay63/1
  in82_repeat/1 -> crp_temp_shared5/3(in2)
  in55_repeat/1 -> crp_temp_shared3/8(in7)
  Delay182/1 -> Delay192/1, in80_repeat/1
  Gain6_out_dtc3/1 -> Add53/2
  Delay152/1 -> in83_repeat/1, Delay162/1
  Delay9/1 -> in39_repeat/1, Delay10/1
  in50_repeat/1 -> crp_temp_shared3/3(in2)
  Delay73/1 -> in16_repeat/1, Delay83/1
  crp_temp_shared3/14(out13) -> Gain13_out_dtc2/1
  Delay222/1 -> Delay232/1, in51_repeat/1
  crp_temp_shared2/1(out0) -> Gain17_out_dtc1/1
  in29_repeat/1 -> crp_temp_shared1/14(in13)
  in0_repeat/1 -> crp_temp_shared/1(in0)
  Delay_Switch/1 -> Delay3_lowered/1
  Logical Operator/1 -> Switch1/2, Switch/2
  Delay19/1 -> in29_repeat/1, Delay20/1
  HFMA1/1(P_theta) -> Add_stage2/1
  Delay233/1 -> in75_repeat/1
  Constant1/1 -> HFMA1/6(F0 Index)
  crp_temp_shared2/2(out1) -> Gain16_out_dtc1/1
  Gain7_out_dtc2/1 -> Add62/2
  Delay14/1 -> in22_repeat/1, Delay24/1
  FixPt Sum11/1 -> FixPt Switch1/3, FixPt Switch1/2
  Gain17_out_dtc3/1 -> Add163/2
  in2_repeat1/1 -> delayMatch4/1, delayMatch1/1
  Delay211/1 -> in27_repeat/1, Delay221/1
  Gain21_out_dtc1/1 -> Add201/2
  Delay203/1 -> in3_repeat/1, Delay214/1
  Delay91/1 -> Delay101/1, in64_repeat/1
  Delay82/1 -> Delay92/1, in90_repeat/1
  Delay81/1 -> Delay91/1, in65_repeat/1
  Delay8/1 -> in40_repeat/1, Delay9/1
  crp_temp_shared/13(out12) -> Gain12_out_dtc/1
  Delay72/1 -> Delay82/1, in91_repeat/1
  crp_temp_shared5/3(out2) -> Gain17_out_dtc3/1
  Delay61/1 -> in67_repeat/1, Delay71/1
  Delay7/1 -> Delay8/1, in41_repeat/1
  crp_temp_shared5/2(out1) -> Gain18_out_dtc3/1
  Delay63/1 -> in17_repeat/1, Delay73/1
  crp_temp_shared5/1(out0) -> Gain19_out_dtc3/1
  Delay51/1 -> Delay61/1, in68_repeat/1
  Delay41/1 -> Delay51/1, in69_repeat/1
  Delay_absorbed/1 -> in2_repeat1/1
  Delay31/1 -> in45_repeat/1, Delay4/1
  Delay213/1 -> Delay223/1, in77_repeat/1
  Delay212/1 -> in52_repeat/1, Delay222/1
  in5_repeat/1 -> crp_temp_shared/6(in5)
  Delay20/1 -> Delay211/1, in28_repeat/1
  crp_temp_shared3/10(out9) -> Gain17_out_dtc2/1
  Delay24/1 -> in21_repeat/1, Delay34/1
  Delay18/1 -> in30_repeat/1, Delay19/1
  Delay173/1 -> in6_repeat/1, Delay183/1
  in42_repeat/1 -> crp_temp_shared2/11(in10)
  Delay16/1 -> Delay17/1, in32_repeat/1
  Delay15/1 -> Delay16/1, in33_repeat/1
  Delay132/1 -> in60_repeat/1, Delay142/1
  Delay102/1 -> Delay113/1, in88_repeat/1
  Delay101/1 -> in63_repeat/1, Delay112/1
  crp_temp_shared2/6(out5) -> Gain12_out_dtc1/1
  Delay/1 -> Delay11/1, in48_repeat/1
  in99_repeat/1 -> crp_temp_shared6/4(in3)
  Gain24_out_dtc2/1 -> Add232/2
  in98_repeat/1 -> crp_temp_shared6/3(in2)
  in93_repeat/1 -> crp_temp_shared5/14(in13)
  in95_repeat/1 -> crp_temp_shared5/16(in15)
  in64_repeat/1 -> crp_temp_shared4/1(in0)
  in92_repeat/1 -> crp_temp_shared5/13(in12)
  crp_temp_shared/2(out1) -> Gain23_out_dtc/1
  in94_repeat/1 -> crp_temp_shared5/15(in14)
  in48_repeat/1 -> crp_temp_shared3/1(in0)
  Gain6_out_dtc/1 -> Add5/2
  in67_repeat/1 -> crp_temp_shared4/4(in3)
  crp_temp_shared5/7(out6) -> Gain13_out_dtc3/1
  in91_repeat/1 -> crp_temp_shared5/12(in11)
  in74_repeat/1 -> crp_temp_shared4/11(in10)
  crp_temp_shared2/10(out9) -> Gain8_out_dtc1/1
  in83_repeat/1 -> crp_temp_shared5/4(in3)
  crp_temp_shared1/11(out10) -> Gain23_out_dtc1/1
  Gain16_out_dtc3/1 -> Add153/2
  in87_repeat/1 -> crp_temp_shared5/8(in7)
  in71_repeat/1 -> crp_temp_shared4/8(in7)
  in86_repeat/1 -> crp_temp_shared5/7(in6)
  crp_temp_shared4/1(out0) -> Gain10_out_dtc2/1
  crp_temp_shared/6(out5) -> Gain19_out_dtc/1
  in70_repeat/1 -> crp_temp_shared4/7(in6)
  Gain22_out_dtc/1 -> Add21/2
  in85_repeat/1 -> crp_temp_shared5/6(in5)
  crp_temp_shared6/2(out1) -> Gain2_out_dtc3/1
  Gain11_out_dtc3/1 -> Add103/2
  in6_repeat/1 -> crp_temp_shared/7(in6)
  in69_repeat/1 -> crp_temp_shared4/6(in5)
  crp_temp_shared4/6(out5) -> Gain5_out_dtc2/1
  in79_repeat/1 -> crp_temp_shared4/16(in15)
  crp_temp_shared5/11(out10) -> Gain9_out_dtc3/1
  Gain24_out_dtc3/1 -> Add233/2
  Gain3_out_dtc3/1 -> Add28/2
  crp_temp_shared5/15(out14) -> Gain5_out_dtc3/1
  crp_temp_shared/8(out7) -> Gain17_out_dtc/1
  in68_repeat/1 -> crp_temp_shared4/5(in4)
  in66_repeat/1 -> crp_temp_shared4/3(in2)
  crp_temp_shared5/13(out12) -> Gain7_out_dtc3/1
  crp_temp_shared5/8(out7) -> Gain12_out_dtc3/1
  in65_repeat/1 -> crp_temp_shared4/2(in1)
  crp_temp_shared5/12(out11) -> Gain8_out_dtc3/1
  crp_temp_shared5/10(out9) -> Gain10_out_dtc3/1
  crp_temp_shared1/15(out14) -> Gain19_out_dtc1/1
  in57_repeat/1 -> crp_temp_shared3/10(in9)
  crp_temp_shared5/5(out4) -> Gain15_out_dtc3/1
  in47_repeat/1 -> crp_temp_shared2/16(in15)
  in46_repeat/1 -> crp_temp_shared2/15(in14)
  Gain15_out_dtc3/1 -> Add143/2
  in77_repeat/1 -> crp_temp_shared4/14(in13)
  in28_repeat/1 -> crp_temp_shared1/13(in12)
  crp_temp_shared2/11(out10) -> Gain7_out_dtc1/1
  crp_temp_shared4/16(out15) -> Gain20_out_dtc3/1
  crp_temp_shared3/4(out3) -> Gain23_out_dtc2/1
  crp_temp_shared4/9(out8) -> Gain2_out_dtc2/1
  Gain19_out_dtc2/1 -> Add182/2
  crp_temp_shared4/13(out12) -> Gain23_out_dtc3/1
  in30_repeat/1 -> crp_temp_shared1/15(in14)
  crp_temp_shared4/12(out11) -> Gain24_out_dtc3/1
  Gain8_out_dtc2/1 -> Add72/2
  crp_temp_shared3/9(out8) -> Gain18_out_dtc2/1
  in33_repeat/1 -> crp_temp_shared2/2(in1)
  Gain20_out_dtc3/1 -> Add193/2
  Gain4_out_dtc2/1 -> Add32/2
  Gain12_out_dtc3/1 -> Add114/2
  Gain5_out_dtc2/1 -> Add42/2
  in58_repeat/1 -> crp_temp_shared3/11(in10)
  in3_repeat/1 -> crp_temp_shared/4(in3)
  Add221/1 -> Add231/1
  crp_temp_shared1/12(out11) -> Gain22_out_dtc1/1
  Gain23_out_dtc3/1 -> Add223/2
  Gain19_out_dtc/1 -> Add18/2
  in56_repeat/1 -> crp_temp_shared3/9(in8)
  in21_repeat/1 -> crp_temp_shared1/6(in5)
  in37_repeat/1 -> crp_temp_shared2/6(in5)
  delayMatch5/1 -> Switch1/1
  in36_repeat/1 -> crp_temp_shared2/5(in4)
  in1_repeat/1 -> crp_temp_shared/2(in1)
  in54_repeat/1 -> crp_temp_shared3/7(in6)
  in63_repeat/1 -> crp_temp_shared3/16(in15)
  in20_repeat/1 -> crp_temp_shared1/5(in4)
  in39_repeat/1 -> crp_temp_shared2/8(in7)
  Gain11_out_dtc1/1 -> Add101/2
  in53_repeat/1 -> crp_temp_shared3/6(in5)
  in62_repeat/1 -> crp_temp_shared3/15(in14)
  in18_repeat/1 -> crp_temp_shared1/3(in2)
  in34_repeat/1 -> crp_temp_shared2/3(in2)
  in52_repeat/1 -> crp_temp_shared3/5(in4)
  in17_repeat/1 -> crp_temp_shared1/2(in1)
  Delay3_lowered/1 -> Delay_Switch/3, bypass_out/1
  crp_temp_shared3/12(out11) -> Gain15_out_dtc2/1
  in15_repeat/1 -> crp_temp_shared/16(in15)
  in16_repeat/1 -> crp_temp_shared1/1(in0)
  crp_temp_shared2/14(out13) -> Gain4_out_dtc1/1
  crp_temp_shared2/9(out8) -> Gain9_out_dtc1/1
  crp_temp_shared2/5(out4) -> Gain13_out_dtc1/1
  crp_temp_shared2/13(out12) -> Gain5_out_dtc1/1
  crp_temp_shared2/4(out3) -> Gain14_out_dtc1/1
  crp_temp_shared1/4(out3) -> Gain5_out_dtc/1
  Gain4_out_dtc1/1 -> Add31/2
  Gain5_out_dtc1/1 -> Add41/2
  in14_repeat/1 -> crp_temp_shared/15(in14)
  Gain18_out_dtc2/1 -> Add172/2
  Gain6_out_dtc1/1 -> Add51/2
  Add223/1 -> Add233/1
  Gain20_out_dtc2/1 -> Add192/2
  Gain23_out_dtc2/1 -> Add222/2
  Gain9_out_dtc1/1 -> Add81/2
  crp_temp_shared1/13(out12) -> Gain21_out_dtc1/1
  crp_temp_shared1/14(out13) -> Gain20_out_dtc1/1
  crp_temp_shared1/10(out9) -> Gain24_out_dtc1/1
  crp_temp_shared1/1(out0) -> Gain8_out_dtc/1
  crp_temp_shared1/5(out4) -> Gain4_out_dtc/1
  crp_temp_shared1/2(out1) -> Gain7_out_dtc/1
  crp_temp_shared/12(out11) -> Gain13_out_dtc/1
  Gain14_out_dtc1/1 -> Add131/2
  in12_repeat/1 -> crp_temp_shared/13(in12)
  in2_repeat/1 -> crp_temp_shared/3(in2)
  crp_temp_shared/7(out6) -> Gain18_out_dtc/1
  crp_temp_shared/15(out14) -> Gain10_out_dtc/1
  crp_temp_shared/10(out9) -> Gain15_out_dtc/1
  crp_temp_shared/5(out4) -> Gain20_out_dtc/1
  crp_temp_shared/4(out3) -> Gain21_out_dtc/1
  Gain23_out_dtc1/1 -> Add221/2
  Gain18_out_dtc/1 -> Add17/2
  Gain24_out_dtc1/1 -> Add231/2
